simulink model "MMC_phase_hackathon_circuit1_HAAS_20260216"  (R2024b)
settings: Solver=FixedStepDiscrete  StartTime=t_init_sim  StopTime=sim_time  FixedStep=Ts  RelTol=1e-3
values from neighbouring files (symbols this model uses):
  a = 1    [param_phase_circuit1_20260216.m]
  C1low1_active = 1    [script_MMC_phase_circuit1_twist_20260216.m]
  C2low1_active = 1    [script_MMC_phase_circuit1_twist_20260216.m]
  C_M_extra = C_m-twist_high_side_C    [param_phase_circuit1_20260216.m]
  duty_cycle = 0.95    [script_MMC_phase_circuit1_twist_20260216.m]
  f0 = 50    [param_phase_circuit1_20260216.m]
  feeder_current_lower_rate_limit = -10    [script_MMC_phase_circuit1_twist_20260216.m]    (also in twist_parameters.m = -500)
  feeder_current_tab = [0.328 0.217 0.162 0.132 0.109 0.094 0.083 0.075 0.068 0.062 0.058 0.054 ... (42 elements, 14x3)]    [feeder_current.mat]
  feeder_current_upper_rate_limit = 0.386/(20e-3)    (= 19.3)    [twist_parameters.m]
  is6VExternallySupplied = true    [script_MMC_phase_circuit1_twist_20260216.m]
  isFeederJumperOpen = true    [script_MMC_phase_circuit1_twist_20260216.m]
  m = 1    [param_phase_circuit1_20260216.m]
  N = 5    [param_phase_circuit1_20260216.m]
  power_losses = false    [script_MMC_phase_circuit1_twist_20260216.m]
  source_V = 0    [script_MMC_phase_circuit1_twist_20260216.m]
  time_charge = 0.1    [script_MMC_phase_circuit1_twist_20260216.m]
  time_decharge = 0.6    [script_MMC_phase_circuit1_twist_20260216.m]
  Ts = 5e-7    (= 5e-07)    [script_MMC_phase_circuit1_twist_20260216.m]
  twist_data_acquisition_delay = 50e-9    (= 5e-08)    [script_MMC_phase_circuit1_twist_20260216.m]    (also in twist_parameters.m)
  twist_data_sampling_period = 1/twist_freq_data_sampling    (= 5e-05)    [script_MMC_phase_circuit1_twist_20260216.m]    (also in twist_parameters.m)
  twist_dead_time = 200e-9    (= 2e-07)    [twist_parameters.m]
  twist_freq_switching = 200e3    (= 200000)    [twist_parameters.m]
  twist_high_side_adc_R = 1/(1/2e6 + 1/2e6 + 1/(330e3+5.6e3))    (= 251272.836178)    [twist_parameters.m]
  twist_high_side_C = 33e-6*4 + 4.7e-6*12    (= 0.0001884)    [twist_parameters.m]
  twist_high_side_feeder_R = 47e3+4.7e3    (= 51700)    [twist_parameters.m]
  twist_high_side_rC = 0.1    [twist_parameters.m]
  twist_low_side_adc_R = 150e3+470    (= 150470)    [twist_parameters.m]
  twist_low_side_C_ceramic = 3*4.7e-6    (= 1.41e-05)    [twist_parameters.m]
  twist_low_side_C_electrolytic = 47e-6    (= 4.7e-05)    [twist_parameters.m]
  twist_low_side_L = 33e-6    (= 3.3e-05)    [twist_parameters.m]
  twist_low_side_rC = 700e-3    (= 0.7)    [twist_parameters.m]
  twist_low_side_rL = 20e-3    (= 0.02)    [twist_parameters.m]
  twist_R_VCC = (tau_VCC/twist_high_side_C  - twist_high_side_rC)/(1-(tau_VCC/twist_high_side_C - twist_high_side_rC)/R_parallel)    (= 1110.74997822)    [twist_parameters.m]
  VDC = 48    [param_phase_circuit1_20260216.m]
undefined symbols (not defined in the file or in its folder): feeder_current, gcbh, sps_rtmsupport, twist_low_side_lC
libraries: spsSeriesRLCBranchLib x130, spsTriangleGeneratorLib x60, spsMosfetLib x60, spsVoltageMeasurementLib x55, spsCurrentMeasurementLib x42, spsControlledCurrentSourceLib x30, spsDiodeLib x22, spsIdealSwitchLib x20, spsControlledVoltageSourceLib x2, spsGroundLib x1, spsMeanLib x1, spspowerguiLib x1
(part 1 of 18)
settings Model: Creator=ana  LastModifiedBy=ana

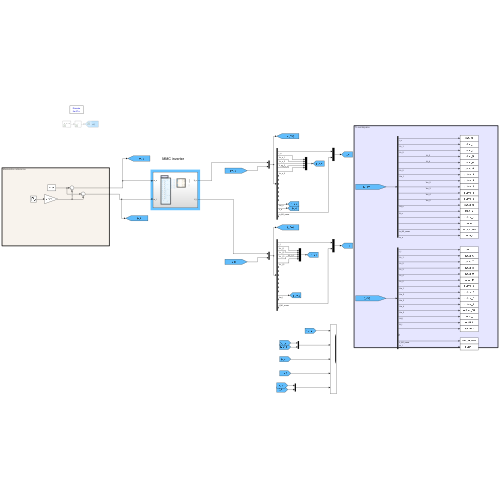
[thumbnail: Simulink's stored preview of the top-level diagram]
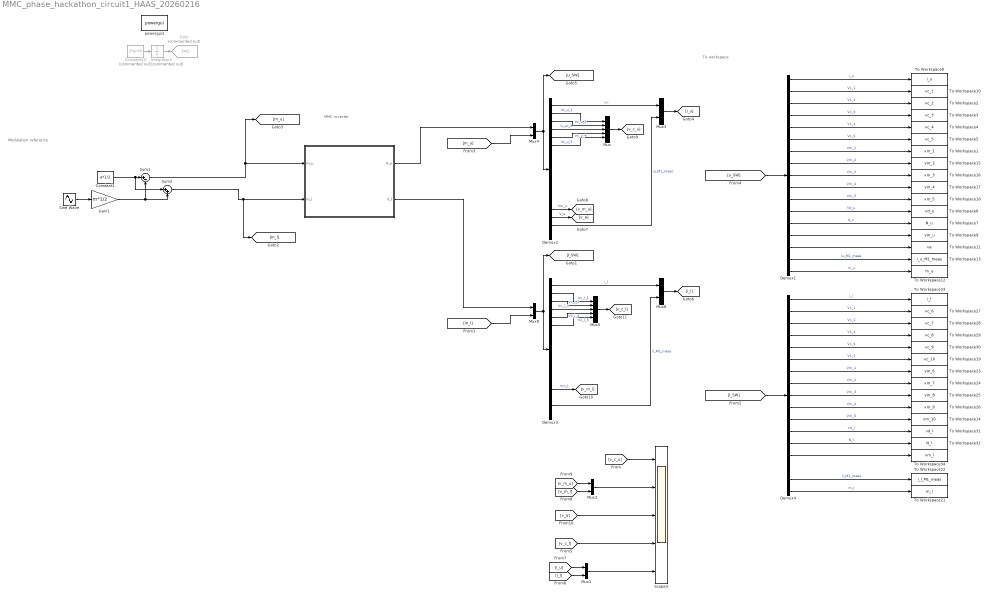
== system MMC_phase_hackathon_circuit1_HAAS_20260216 ==
  note: MMC inverter
  note: To workspace
  note: Modulation reference
  " " : Subsystem
  Constant1 : Constant  Value=a*1/2
  Constant12 : Constant  Commented=on  Value=2*pi*f0
  Demux{1..4} (4 alike) : Demux  Outputs=17
  Gain1 : Gain  Gain=m*1/2
  Goto : Goto  Commented=on  GotoTag=wt
  Integrator2 : Integrator  Commented=on
  Mux : Mux  Inputs=5
  Mux{1..4,8..9} (6 alike) : Mux  Inputs=2
  Mux5 : Mux  Inputs=5
  Scope3 : Scope  NumInputPorts=5
  Sine Wave : Sin  Frequency=2*pi*f0  SampleTime=Ts
  Sum1 : Sum  Inputs=|+-
  Sum2 : Sum  Inputs=|++
  To Workspace1 : ToWorkspace  VariableName=vm_1  SaveFormat=Structure With Time  SampleTime=-1
  To Workspace10 : ToWorkspace  VariableName=vc_1  SaveFormat=Structure With Time  SampleTime=-1
  To Workspace11 : ToWorkspace  VariableName=va  SaveFormat=Structure With Time  SampleTime=-1
  To Workspace12 : ToWorkspace  VariableName=m_u  SaveFormat=Structure With Time  SampleTime=-1
  To Workspace13 : ToWorkspace  VariableName=i_u_M1_meas  SaveFormat=Structure With Time  SampleTime=-1
  To Workspace14 : ToWorkspace  VariableName=vm_10  SaveFormat=Structure With Time  SampleTime=-1
  To Workspace15 : ToWorkspace  VariableName=vm_2  SaveFormat=Structure With Time  SampleTime=-1
  To Workspace16 : ToWorkspace  VariableName=vm_3  SaveFormat=Structure With Time  SampleTime=-1
  To Workspace17 : ToWorkspace  VariableName=vm_4  SaveFormat=Structure With Time  SampleTime=-1
  To Workspace18 : ToWorkspace  VariableName=vm_5  SaveFormat=Structure With Time  SampleTime=-1
  To Workspace19 : ToWorkspace  VariableName=vc_10  SaveFormat=Structure With Time  SampleTime=-1
  To Workspace2 : ToWorkspace  VariableName=vc_2  SaveFormat=Structure With Time  SampleTime=-1
  To Workspace21 : ToWorkspace  VariableName=m_l  SaveFormat=Structure With Time  SampleTime=-1
  To Workspace22 : ToWorkspace  VariableName=i_l_M1_meas  SaveFormat=Structure With Time  SampleTime=-1
  To Workspace23 : ToWorkspace  VariableName=vm_6  SaveFormat=Structure With Time  SampleTime=-1
  To Workspace24 : ToWorkspace  VariableName=vm_7  SaveFormat=Structure With Time  SampleTime=-1
  To Workspace25 : ToWorkspace  VariableName=vm_8  SaveFormat=Structure With Time  SampleTime=-1
  To Workspace26 : ToWorkspace  VariableName=vm_9  SaveFormat=Structure With Time  SampleTime=-1
  To Workspace27 : ToWorkspace  VariableName=vc_6  SaveFormat=Structure With Time  SampleTime=-1
  To Workspace28 : ToWorkspace  VariableName=vc_7  SaveFormat=Structure With Time  SampleTime=-1
  To Workspace29 : ToWorkspace  VariableName=vc_8  SaveFormat=Structure With Time  SampleTime=-1
  To Workspace3 : ToWorkspace  VariableName=vc_3  SaveFormat=Structure With Time  SampleTime=-1
  To Workspace30 : ToWorkspace  VariableName=vc_9  SaveFormat=Structure With Time  SampleTime=-1
  To Workspace31 : ToWorkspace  VariableName=vd_l  SaveFormat=Structure With Time  SampleTime=-1
  To Workspace32 : ToWorkspace  VariableName=N_l  SaveFormat=Structure With Time  SampleTime=-1
  To Workspace33 : ToWorkspace  VariableName=i_l  SaveFormat=Structure With Time  SampleTime=-1
  To Workspace34 : ToWorkspace  VariableName=vm_l  SaveFormat=Structure With Time  SampleTime=-1
  To Workspace4 : ToWorkspace  VariableName=vc_4  SaveFormat=Structure With Time  SampleTime=-1
  To Workspace5 : ToWorkspace  VariableName=vc_5  SaveFormat=Structure With Time  SampleTime=-1
  To Workspace6 : ToWorkspace  VariableName=vd_u  SaveFormat=Structure With Time  SampleTime=-1
  To Workspace7 : ToWorkspace  VariableName=N_u  SaveFormat=Structure With Time  SampleTime=-1
  To Workspace8 : ToWorkspace  VariableName=i_u  SaveFormat=Structure With Time  SampleTime=-1
  To Workspace9 : ToWorkspace  VariableName=vm_u  SaveFormat=Structure With Time  SampleTime=-1
  powergui1 : spspowerguiLib/powergui  Priority=1  SimulationMode=Discrete  SampleTime=Ts  frequency=60  Iterations=50  frequencyindice=0  Pbase=100e6  ErrMax=1e-4  UnitsV=V  UnitsW=W  buscounter=0  FunctionMessages=off  echomessages=off  EnableUseOfTLC=off  CurrentSourceSwitches=off  DisableSnubberDevices=off  DisableRonSwitches=off  DisableVfSwitches=off  DisplayEquations=off  AutomaticDiscreteSolvers=off  SolverType=Backward Euler  Interpol=off  ExternalGateDelay=off  methode=off  Ts=0  x0status=blocks  SPID=off  SwTol=0  HookPort=off  NonlinearTolerance=1e-4  nMaxIteration=100  ContinueOnMaxIteration=off  RestoreLinks=warning  ResistiveCurrentMeasurement=off  Frange=[0:2:500]  Ylog=off  Xlog=on  ShowGrid=off  save=off  variable=ZData  structure=0  ZoomFFT=off  StartTime=0.0  cycles=1  DisplayStyle=1  fundamental=60  FreqAxis=off  MaxFrequency=1000  frequencyindicesteady=1  RmsSteady=1  display=off
  wires:
  [u_SW] -> Demux1/1
  Demux1/8 -> To Workspace15/1  "Vm_2"
  Demux1/17 -> To Workspace12/1  "m_u"
  Demux1/10 -> To Workspace17/1  "Vm_4"
  Demux1/5 -> To Workspace4/1  "Vc_4"
  Demux1/12 -> To Workspace6/1  "Vd_u"
  " "/1(X_u) -> Mux4/1
  Demux2/1 -> Mux3/1  "i_u"
  Constant1/1 -> Sum2/1, Sum1/1
  Demux1/11 -> To Workspace18/1  "Vm_5"
  [m_u] -> Mux4/2
  Demux2/6 -> Mux/5  "Vc_u_5"
  Mux4/1 -> [u_SW], Demux2/1
  Constant12/1 -> Integrator2/1
  Integrator2/1 -> Goto/1
  Demux1/9 -> To Workspace16/1  "Vm_3"
  Demux1/7 -> To Workspace1/1  "Vm_1"
  Demux1/3 -> To Workspace2/1  "Vc_2"
  Demux1/4 -> To Workspace3/1  "Vc_3"
  Demux1/6 -> To Workspace5/1  "Vc_5"
  Gain1/1 -> Sum1/2, Sum2/2
  Demux1/2 -> To Workspace10/1  "Vc_1"
  Demux2/2 -> Mux/1  "Vc_u_1"
  Demux1/1 -> To Workspace8/1  "i_u"
  Demux2/5 -> Mux/4  "Vc_u_4"
  Demux2/3 -> Mux/2  "Vc_u_2"
  Demux2/4 -> Mux/3  "V_uc_3"
  Sum1/1 -> [m_u], " "/1(m_u)
  Demux2/14 -> [v_m_u]  "Vm_u"
  Sine Wave/1 -> Gain1/1
  Demux1/13 -> To Workspace7/1  "N_u"
  Demux1/14 -> To Workspace9/1
  Demux1/15 -> To Workspace11/1
  Demux2/16 -> Mux3/2  "iu_M1_meas"
  Demux1/16 -> To Workspace13/1  "iu_M1_meas"
  Sum2/1 -> [m_l], " "/2(m_l)
  Demux3/6 -> Mux5/5  "Vc_l_5"
  Mux8/1 -> [i_l]
  Mux9/1 -> [l_SW], Demux3/1
  Demux3/2 -> Mux5/1  "Vc_l_1"
  Demux3/3 -> Mux5/2  "Vc_l_2"
  Demux3/1 -> Mux8/1  "i_l"
  [m_l] -> Mux9/2
  " "/2(X_l) -> Mux9/1
  Demux3/14 -> [v_m_l]  "Vm_l"
  Demux3/16 -> Mux8/2  "il_M1_meas"
  Demux3/5 -> Mux5/4  "Vc_l_4"
  Demux3/4 -> Mux5/3  "Vc_l_3"
  Demux4/2 -> To Workspace27/1  "Vc_1"
  Demux4/12 -> To Workspace31/1  "Vd_l"
  Demux4/17 -> To Workspace21/1  "m_l"
  [l_SW] -> Demux4/1
  Demux4/1 -> To Workspace33/1  "i_l"
  Demux4/13 -> To Workspace32/1  "N_l"
  Demux4/14 -> To Workspace34/1
  Demux4/16 -> To Workspace22/1  "il_M1_meas"
  Demux4/3 -> To Workspace28/1  "Vc_2"
  Demux4/4 -> To Workspace29/1  "Vc_3"
  Demux4/5 -> To Workspace30/1  "Vc_4"
  Demux4/6 -> To Workspace19/1  "Vc_5"
  Demux4/7 -> To Workspace23/1  "Vm_1"
  Demux4/8 -> To Workspace24/1  "Vm_2"
  Demux4/9 -> To Workspace25/1  "Vm_3"
  Demux4/10 -> To Workspace26/1  "Vm_4"
  Demux4/11 -> To Workspace14/1  "Vm_5"
  Mux3/1 -> [i_u]
  Demux2/15 -> [v_a]  "V_a"
  Mux/1 -> [v_c_u]
  Mux5/1 -> [v_c_l]
  [v_c_u] -> Scope3/1
  [i_u] -> Mux1/1
  [i_l] -> Mux1/2
  [v_m_u] -> Mux2/1
  [v_m_l] -> Mux2/2
  [v_a] -> Scope3/3
  Mux2/1 -> Scope3/2
  Mux1/1 -> Scope3/5
  [v_c_l] -> Scope3/4

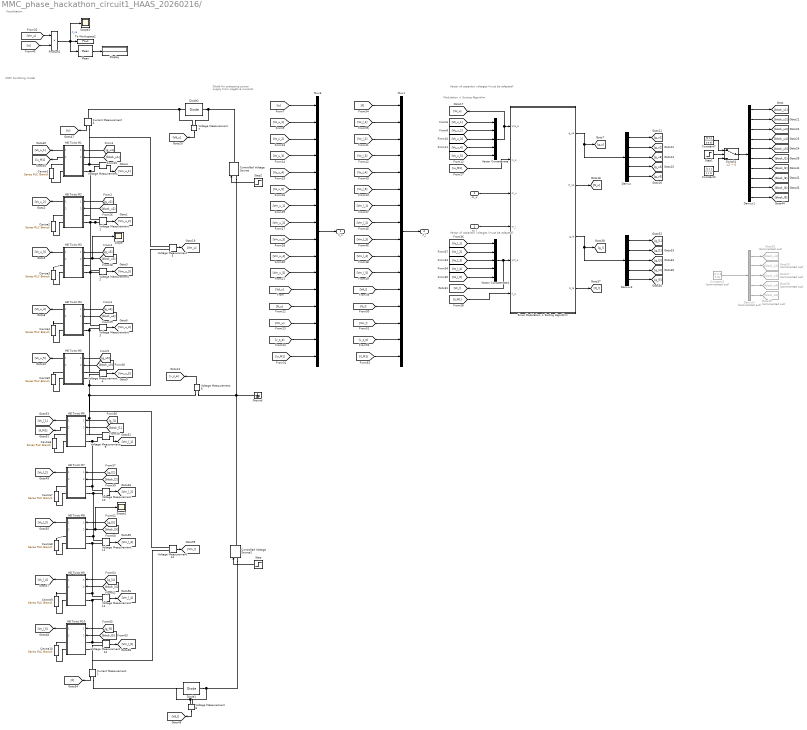
== system MMC_phase_hackathon_circuit1_HAAS_20260216/  ==
  note: Vector of capacitor voltages (must be adapted)
  note: Visualisation
  note: Modulation + Sorting Algorithm
  note: MMC Switching model
  note: Diode for protecting power supply from negative currents
  note: Vector of capacitor voltages (must be adapted)
  m_u : Inport
  m_l : Inport  Port=2
  Cextra{1..10} (10 alike) : spsSeriesRLCBranchLib/Series RLC Branch  LConnTagsString=__new0  RConnTagsString=__new0  BranchType=C  Resistance=twist_high_side_rC  Inductance=1e-3  SetiL0=off  InitialCurrent=0  Capacitance=C_M_extra  Setx0=on  InitialVoltage=source_V  Measurements=None
  Constant2 : Constant  Value=[1 1 1 1 1 1 1 1 1 1]
  Constant3 : Constant  Commented=on  Value=[0 0 0 0 0]
  Constant7 : Constant  Value=[0 0 0 0 0 0 0 0 0 0]
  Controlled Voltage Source : spsControlledVoltageSourceLib/Controlled Voltage Source  Initialize=on  Source_Type=DC  Amplitude=0  Phase=0  Frequency=0  Measurements=None
  Controlled Voltage Source1 : spsControlledVoltageSourceLib/Controlled Voltage Source  Initialize=on  Source_Type=DC  Amplitude=0  Phase=0  Frequency=0  Measurements=None
  Current Measurement1 : spsCurrentMeasurementLib/Current Measurement  PhasorSimulation=off  OutputType=Complex  PSBequivalent=0
  Current Measurement4 : spsCurrentMeasurementLib/Current Measurement  PhasorSimulation=off  OutputType=Complex  PSBequivalent=0
  Demux : Demux  Outputs=5
  Demux1 : Demux  Outputs=10
  Demux2 : Demux  Commented=on  Outputs=5
  Demux3 : Demux  Outputs=5
  Diode1 : spsDiodeLib/Diode  Ron=0.001  Lon=0  Vf=0.8  IC=0  UseSnubber=0  Rs=1e5  Cs=inf  Measurements=off
  Diode2 : spsDiodeLib/Diode  Ron=0.001  Lon=0  Vf=0.8  IC=0  UseSnubber=0  Rs=1e5  Cs=inf  Measurements=off
  Display : Display
  Goto25 : Goto  Commented=on  GotoTag=block_u1
  Goto26 : Goto  Commented=on  GotoTag=block_u2
  Goto27 : Goto  Commented=on  GotoTag=block_u3
  Goto28 : Goto  Commented=on  GotoTag=block_u4
  Goto29 : Goto  Commented=on  GotoTag=block_u5
  Ground : spsGroundLib/Ground  LConnTagsString=a
  HB Twist M1 : Subsystem
  HB Twist M10 : Subsystem
  HB Twist M2 : Subsystem
  HB Twist M3 : Subsystem
  HB Twist M4 : Subsystem
  HB Twist M5 : Subsystem
  HB Twist M6 : Subsystem
  HB Twist M7 : Subsystem
  HB Twist M8 : Subsystem
  HB Twist M9 : Subsystem
  Mean : spsMeanLib/Mean  Freq=f0  Vinit=0  Ts=Ts
  Mux1 : Mux  Inputs=16
  Mux6 : Mux  Inputs=16
  Product1 : Product
  Scope : Scope
  Scope1 : Scope
  Scope3 : Scope
  Sinus Modulation + Sorting Algorithm : Subsystem
  Step : Step  Time=time_decharge  Before=VDC/2  After=0  SampleTime=0
  Step1 : Step  Time=time_charge  SampleTime=Ts
  Step2 : Step  Time=time_decharge  Before=VDC/2  After=0  SampleTime=0
  Switch1 : Switch  Criteria=u2 > Threshold  SaturateOnIntegerOverflow=off  InputSameDT=off
  To Workspace2 : ToWorkspace  VariableName=Pout  SaveFormat=Structure With Time  SampleTime=-1
  Vector Concatenate : Concatenate  NumInputs=5
  Vector Concatenate1 : Concatenate  NumInputs=5
  Voltage Measurement{,1..14} (15 alike) : spsVoltageMeasurementLib/Voltage Measurement  PhasorSimulation=off  OutputType=Complex  PSBequivalent=0
  X_u : Outport
  X_l : Outport  Port=2
  wires:
  [Vc_u_1] -> Mux6/2
  Mux6/1 -> X_u/1
  Current Measurement4/1 -> [iu]
  Sinus Modulation + Sorting Algorithm/1(g_ua) -> Demux/1, [g_u]
  [iu_M1] -> Sinus Modulation + Sorting Algorithm/2(iu_a)
  Vector Concatenate/1 -> [Vc_u], Sinus Modulation + Sorting Algorithm/1(Vcu_a)
  m_u/1 -> Sinus Modulation + Sorting Algorithm/3(m_u)
  Product1/1 -> Mean/1, Scope3/1, To Workspace2/1  "P_sa"
  Voltage Measurement6/1 -> [v_s_a]
  [iu] -> Product1/2
  HB Twist M1/1(v_High) -> [Vc_u_1]
  Voltage Measurement/1 -> [Vm_u_1]
  [g_u1] -> HB Twist M1/1(duty_cycle1)
  Voltage Measurement1/1 -> [Vm_u_2]
  HB Twist M2/1(v_High) -> [Vc_u_2]
  [g_u2] -> HB Twist M2/1(duty_cycle1)
  [g_u3] -> HB Twist M3/1(duty_cycle1)
  HB Twist M3/1(v_High) -> [Vc_u_3]
  Voltage Measurement2/1 -> [Vm_u_3]
  [g_u4] -> HB Twist M4/1(duty_cycle1)
  HB Twist M4/1(v_High) -> [Vc_u_4]
  Voltage Measurement3/1 -> [Vm_u_4]
  [g_u5] -> HB Twist M5/1(duty_cycle1)
  HB Twist M5/1(v_High) -> [Vc_u_5]
  Voltage Measurement4/1 -> [Vm_u_5]
  [Vc_u_1] -> Vector Concatenate/1
  [Vc_u_2] -> Vector Concatenate/2
  [Vc_u_3] -> Vector Concatenate/3
  [Vc_u_4] -> Vector Concatenate/4
  [Vc_u_5] -> Vector Concatenate/5
  Demux/1 -> [g_u1]
  Demux/2 -> [g_u2]
  Demux/3 -> [g_u3]
  Demux/4 -> [g_u4]
  Demux/5 -> [g_u5]
  [iu] -> Mux6/1
  [Vc_u_2] -> Mux6/3
  [Vc_u_3] -> Mux6/4
  [Vc_u_4] -> Mux6/5
  [Vc_u_5] -> Mux6/6
  [Vm_u_1] -> Mux6/7
  [Vm_u_2] -> Mux6/8
  [Vm_u_3] -> Mux6/9
  [Vm_u_4] -> Mux6/10
  [Vm_u_5] -> Mux6/11
  [Vd_u] -> Mux6/12
  Sinus Modulation + Sorting Algorithm/2(N_ua) -> [N_u]
  [N_u] -> Mux6/13
  Voltage Measurement5/1 -> [Vm_u]
  [Vm_u] -> Mux6/14
  [v_s_a] -> Mux6/15
  Voltage Measurement7/1 -> [Vd_u]
  Mean/1 -> Display/1
  [block_u1] -> HB Twist M1/2(block_leg1)
  [block_u2] -> HB Twist M2/2(block_leg1)
  [block_u3] -> HB Twist M3/2(block_leg1), Scope/1
  [block_u4] -> HB Twist M4/2(block_leg1)
  [block_u5] -> HB Twist M5/2(block_leg1)
  Step1/1 -> Switch1/2
  Switch1/1 -> Demux1/1
  Demux1/1 -> [block_u1]
  Demux1/2 -> [block_u2]
  Demux1/3 -> [block_u3]
  Demux1/4 -> [block_u4]
  Demux1/5 -> [block_u5]
  Constant7/1 -> Switch1/1
  Constant2/1 -> Switch1/3
  Demux2/3 -> Goto27/1
  Demux2/4 -> Goto28/1
  Constant3/1 -> Demux2/1
  Demux2/5 -> Goto29/1
  Demux2/2 -> Goto26/1
  Demux2/1 -> Goto25/1
  HB Twist M1/2(i_1Low) -> [iu_M1]
  [iu_M1] -> Mux6/16
  [Vm_u] -> Product1/1
  m_l/1 -> Sinus Modulation + Sorting Algorithm/4(m_l)
  Vector Concatenate1/1 -> Sinus Modulation + Sorting Algorithm/5(Vcl_a), [Vc_l]
  [Vc_l_1] -> Vector Concatenate1/1
  [Vc_l_2] -> Vector Concatenate1/2
  [Vc_l_3] -> Vector Concatenate1/3
  [Vc_l_4] -> Vector Concatenate1/4
  [Vc_l_5] -> Vector Concatenate1/5
  [il_M1] -> Sinus Modulation + Sorting Algorithm/6(il_a)
  Sinus Modulation + Sorting Algorithm/3(g_la) -> Demux3/1, [g_l]
  Demux3/4 -> [g_l4]
  Demux3/3 -> [g_l3]
  Demux3/5 -> [g_l5]
  Demux3/2 -> [g_l2]
  Sinus Modulation + Sorting Algorithm/4(N_la) -> [N_l]
  Demux3/1 -> [g_l1]
  Demux1/6 -> [block_l1]
  Demux1/7 -> [block_l2]
  Demux1/8 -> [block_l3]
  Demux1/9 -> [block_l4]
  Demux1/10 -> [block_l5]
  [il] -> Mux1/1
  [Vc_l_5] -> Mux1/6
  [Vc_l_1] -> Mux1/2
  Mux1/1 -> X_l/1
  [Vm_l_4] -> Mux1/10
  [Vc_l_4] -> Mux1/5
  [Vm_l_2] -> Mux1/8
  [Vm_l_5] -> Mux1/11
  [il_M1] -> Mux1/16
  [Vc_l_2] -> Mux1/3
  [Vd_l] -> Mux1/12
  [Vm_l_1] -> Mux1/7
  [Vm_l_3] -> Mux1/9
  [Vm_l] -> Mux1/14
  [Vc_l_3] -> Mux1/4
  [N_l] -> Mux1/13
  [v_s_a] -> Mux1/15
  Voltage Measurement8/1 -> [Vd_l]
  Step/1 -> Controlled Voltage Source1/1
  Voltage Measurement12/1 -> [Vm_l_4]
  HB Twist M8/1(v_High) -> [Vc_l_3]
  HB Twist M7/1(v_High) -> [Vc_l_2]
  [block_l2] -> HB Twist M7/2(block_leg1)
  [g_l1] -> HB Twist M6/1(duty_cycle1)
  Voltage Measurement11/1 -> [Vm_l_3]
  Current Measurement1/1 -> [il]
  [g_l3] -> HB Twist M8/1(duty_cycle1)
  HB Twist M10/1(v_High) -> [Vc_l_5]
  [g_l2] -> HB Twist M7/1(duty_cycle1)
  HB Twist M9/1(v_High) -> [Vc_l_4]
  [block_l5] -> HB Twist M10/2(block_leg1)
  [block_l3] -> HB Twist M8/2(block_leg1), Scope1/1
  Voltage Measurement9/1 -> [Vm_l_1]
  Voltage Measurement10/1 -> [Vm_l_2]
  HB Twist M6/1(v_High) -> [Vc_l_1]
  [g_l5] -> HB Twist M10/1(duty_cycle1)
  HB Twist M6/2(i_1Low) -> [il_M1]
  [block_l1] -> HB Twist M6/2(block_leg1)
  [g_l4] -> HB Twist M9/1(duty_cycle1)
  [block_l4] -> HB Twist M9/2(block_leg1)
  Voltage Measurement13/1 -> [Vm_l_5]
  Voltage Measurement14/1 -> [Vm_l]
  Step2/1 -> Controlled Voltage Source/1
  connections:
  Voltage Measurement/LConn1 -- Current Measurement4/RConn1 -- Voltage Measurement5/LConn1 -- HB Twist M1/LConn1
  Voltage Measurement7/LConn2 -- Diode2/RConn1 -- Current Measurement4/LConn1
  Voltage Measurement3/LConn2 -- HB Twist M4/LConn2 -- HB Twist M5/LConn1 -- Voltage Measurement4/LConn1
  HB Twist M1/LConn2 -- Voltage Measurement/LConn2 -- HB Twist M2/LConn1 -- Voltage Measurement1/LConn1
  Voltage Measurement2/LConn2 -- HB Twist M3/LConn2 -- HB Twist M4/LConn1 -- Voltage Measurement3/LConn1
  Voltage Measurement1/LConn2 -- HB Twist M2/LConn2 -- HB Twist M3/LConn1 -- Voltage Measurement2/LConn1
  Voltage Measurement8/LConn1 -- Diode1/LConn1 -- Current Measurement1/RConn1
  Voltage Measurement7/LConn1 -- Diode2/LConn1 -- Controlled Voltage Source/RConn1
  Cextra1/LConn1 -- HB Twist M1/RConn1
  HB Twist M1/RConn2 -- Cextra1/RConn1
  Cextra2/LConn1 -- HB Twist M2/RConn1
  HB Twist M2/RConn2 -- Cextra2/RConn1
  HB Twist M3/RConn1 -- Cextra3/LConn1
  HB Twist M3/RConn2 -- Cextra3/RConn1
  Cextra4/LConn1 -- HB Twist M4/RConn1
  HB Twist M4/RConn2 -- Cextra4/RConn1
  HB Twist M5/RConn1 -- Cextra5/LConn1
  HB Twist M5/RConn2 -- Cextra5/RConn1
  Controlled Voltage Source/LConn1 -- Controlled Voltage Source1/RConn1 -- Voltage Measurement6/LConn2 -- Ground/LConn1
  Controlled Voltage Source1/LConn1 -- Diode1/RConn1 -- Voltage Measurement8/LConn2
  Voltage Measurement4/LConn2 -- Voltage Measurement9/LConn1 -- HB Twist M6/LConn1 -- Voltage Measurement14/LConn1 -- Voltage Measurement6/LConn1 -- Voltage Measurement5/LConn2 -- HB Twist M5/LConn2
  Voltage Measurement13/LConn1 -- HB Twist M10/LConn1 -- Voltage Measurement12/LConn2 -- HB Twist M9/LConn2
  Voltage Measurement11/LConn1 -- HB Twist M8/LConn1 -- Voltage Measurement10/LConn2 -- HB Twist M7/LConn2
  Voltage Measurement10/LConn1 -- HB Twist M6/LConn2 -- Voltage Measurement9/LConn2 -- HB Twist M7/LConn1
  Voltage Measurement13/LConn2 -- Voltage Measurement14/LConn2 -- Current Measurement1/LConn1 -- HB Twist M10/LConn2
  Voltage Measurement12/LConn1 -- HB Twist M9/LConn1 -- Voltage Measurement11/LConn2 -- HB Twist M8/LConn2
  Cextra9/LConn1 -- HB Twist M9/RConn1
  Cextra6/LConn1 -- HB Twist M6/RConn1
  Cextra7/LConn1 -- HB Twist M7/RConn1
  HB Twist M6/RConn2 -- Cextra6/RConn1
  HB Twist M8/RConn1 -- Cextra8/LConn1
  HB Twist M7/RConn2 -- Cextra7/RConn1
  HB Twist M10/RConn2 -- Cextra10/RConn1
  HB Twist M8/RConn2 -- Cextra8/RConn1
  HB Twist M10/RConn1 -- Cextra10/LConn1
  HB Twist M9/RConn2 -- Cextra9/RConn1

== system MMC_phase_hackathon_circuit1_HAAS_20260216/ /HB Twist M1 ==
  duty_cycle1 : Inport
  block_leg1 : Inport  Port=2
  Constant10 : Constant  Value=C2low1_active
  Constant11 : Constant  Value=isFeederJumperOpen
  Constant2 : Constant  Value=feeder_current_tab
  Constant3 : Constant  Value=-0.1
  Constant4 : Constant  Value=is6VExternallySupplied
  Constant5 : Constant  Value=power_losses
  Constant8 : Constant
  Constant9 : Constant  Value=C1low1_active
  Gain : Gain  Gain=-1
  Saturation : Saturate  UpperLimit=1  LowerLimit=0
  Twist Power Block : Subsystem
  Voltage Measurement8 : spsVoltageMeasurementLib/Voltage Measurement  PhasorSimulation=off  OutputType=Complex  PSBequivalent=0
  Load leg1 : PMIOPort  Side=Left
  Load GND : PMIOPort  Port=2  Side=Left
  Vhigh + : PMIOPort  Port=3  Side=Right
  Vhigh GND : PMIOPort  Port=4  Side=Right
  v_High : Outport
  i_1Low : Outport  Port=2
  wires:
  duty_cycle1/1 -> Saturation/1, Twist Power Block/1(duty_cycle1)
  Twist Power Block/2(v1Meas) -> [v1Meas_twist]
  block_leg1/1 -> Twist Power Block/8(block_leg1)
  Constant4/1 -> Twist Power Block/10(is6VExternallySupplied)
  Constant5/1 -> Twist Power Block/7(powerLosses)
  Twist Power Block/1(i1Meas) -> Gain/1
  Twist Power Block/5(v2Meas) -> [v2Meas_twist]
  Constant10/1 -> Twist Power Block/5(C2low_active)
  Constant3/1 -> Twist Power Block/3(duty_cycle2)
  Constant11/1 -> Twist Power Block/11(isFeederJumperOpen)
  Twist Power Block/4(i2Meas) -> [i2Meas_twist]
  Twist Power Block/3(vHMeas) -> [vHMeas_twist]
  Constant9/1 -> Twist Power Block/4(C1low_active)
  Twist Power Block/9(Q2) -> [Q2]
  Constant2/1 -> Twist Power Block/6(feeder_current_tab)
  Twist Power Block/6(iHMeas) -> [iHMeas_twist]
  Twist Power Block/7(feeder_current) -> [feeder_current_twist]
  Constant8/1 -> Twist Power Block/9(block_leg2)
  Twist Power Block/8(Q1) -> [Q1]
  Voltage Measurement8/1 -> v_High/1, [Vc_M1]
  Saturation/1 -> Twist Power Block/2(duty_cycle1_bis)
  Gain/1 -> i_1Low/1, [i1Meas_twist]
  connections:
  Voltage Measurement8/LConn2 -- Vhigh GND/RConn1 -- Twist Power Block/RConn2
  Voltage Measurement8/LConn1 -- Vhigh +/RConn1 -- Twist Power Block/RConn1
  Twist Power Block/LConn3 -- Load GND/RConn1
  Load leg1/RConn1 -- Twist Power Block/LConn1

== system MMC_phase_hackathon_circuit1_HAAS_20260216/ /HB Twist M10 ==
  duty_cycle1 : Inport
  block_leg1 : Inport  Port=2
  Constant10 : Constant  Value=C2low1_active
  Constant11 : Constant  Value=isFeederJumperOpen
  Constant2 : Constant  Value=feeder_current_tab
  Constant3 : Constant  Value=-0.1
  Constant4 : Constant  Value=is6VExternallySupplied
  Constant5 : Constant  Value=power_losses
  Constant8 : Constant
  Constant9 : Constant  Value=C1low1_active
  Gain : Gain  Gain=-1
  Saturation : Saturate  UpperLimit=1  LowerLimit=0
  Twist Power Block : Subsystem
  Voltage Measurement8 : spsVoltageMeasurementLib/Voltage Measurement  PhasorSimulation=off  OutputType=Complex  PSBequivalent=0
  Load leg1 : PMIOPort  Side=Left
  Load GND : PMIOPort  Port=2  Side=Left
  Vhigh + : PMIOPort  Port=3  Side=Right
  Vhigh GND : PMIOPort  Port=4  Side=Right
  v_High : Outport
  i_1Low : Outport  Port=2
  wires:
  duty_cycle1/1 -> Saturation/1, Twist Power Block/1(duty_cycle1)
  Twist Power Block/2(v1Meas) -> [v1Meas_twist]
  block_leg1/1 -> Twist Power Block/8(block_leg1)
  Constant4/1 -> Twist Power Block/10(is6VExternallySupplied)
  Constant5/1 -> Twist Power Block/7(powerLosses)
  Twist Power Block/1(i1Meas) -> Gain/1
  Twist Power Block/5(v2Meas) -> [v2Meas_twist]
  Constant10/1 -> Twist Power Block/5(C2low_active)
  Constant3/1 -> Twist Power Block/3(duty_cycle2)
  Constant11/1 -> Twist Power Block/11(isFeederJumperOpen)
  Twist Power Block/4(i2Meas) -> [i2Meas_twist]
  Twist Power Block/3(vHMeas) -> [vHMeas_twist]
  Constant9/1 -> Twist Power Block/4(C1low_active)
  Twist Power Block/9(Q2) -> [Q2]
  Constant2/1 -> Twist Power Block/6(feeder_current_tab)
  Twist Power Block/6(iHMeas) -> [iHMeas_twist]
  Twist Power Block/7(feeder_current) -> [feeder_current_twist]
  Constant8/1 -> Twist Power Block/9(block_leg2)
  Twist Power Block/8(Q1) -> [Q1]
  Voltage Measurement8/1 -> v_High/1, [Vc_M1]
  Saturation/1 -> Twist Power Block/2(duty_cycle1_bis)
  Gain/1 -> i_1Low/1, [i1Meas_twist]
  connections:
  Voltage Measurement8/LConn2 -- Vhigh GND/RConn1 -- Twist Power Block/RConn2
  Voltage Measurement8/LConn1 -- Vhigh +/RConn1 -- Twist Power Block/RConn1
  Twist Power Block/LConn3 -- Load GND/RConn1
  Load leg1/RConn1 -- Twist Power Block/LConn1

== system MMC_phase_hackathon_circuit1_HAAS_20260216/ /HB Twist M2 ==
  duty_cycle1 : Inport
  block_leg1 : Inport  Port=2
  Constant10 : Constant  Value=C2low1_active
  Constant11 : Constant  Value=isFeederJumperOpen
  Constant2 : Constant  Value=feeder_current_tab
  Constant3 : Constant  Value=-0.1
  Constant4 : Constant  Value=is6VExternallySupplied
  Constant5 : Constant  Value=power_losses
  Constant8 : Constant
  Constant9 : Constant  Value=C1low1_active
  Gain : Gain  Gain=-1
  Saturation : Saturate  UpperLimit=1  LowerLimit=0
  Twist Power Block : Subsystem
  Voltage Measurement8 : spsVoltageMeasurementLib/Voltage Measurement  PhasorSimulation=off  OutputType=Complex  PSBequivalent=0
  Load leg1 : PMIOPort  Side=Left
  Load GND : PMIOPort  Port=2  Side=Left
  Vhigh + : PMIOPort  Port=3  Side=Right
  Vhigh GND : PMIOPort  Port=4  Side=Right
  v_High : Outport
  i_1Low : Outport  Port=2
  wires:
  duty_cycle1/1 -> Saturation/1, Twist Power Block/1(duty_cycle1)
  Twist Power Block/2(v1Meas) -> [v1Meas_twist]
  block_leg1/1 -> Twist Power Block/8(block_leg1)
  Constant4/1 -> Twist Power Block/10(is6VExternallySupplied)
  Constant5/1 -> Twist Power Block/7(powerLosses)
  Twist Power Block/1(i1Meas) -> Gain/1
  Twist Power Block/5(v2Meas) -> [v2Meas_twist]
  Constant10/1 -> Twist Power Block/5(C2low_active)
  Constant3/1 -> Twist Power Block/3(duty_cycle2)
  Constant11/1 -> Twist Power Block/11(isFeederJumperOpen)
  Twist Power Block/4(i2Meas) -> [i2Meas_twist]
  Twist Power Block/3(vHMeas) -> [vHMeas_twist]
  Constant9/1 -> Twist Power Block/4(C1low_active)
  Twist Power Block/9(Q2) -> [Q2]
  Constant2/1 -> Twist Power Block/6(feeder_current_tab)
  Twist Power Block/6(iHMeas) -> [iHMeas_twist]
  Twist Power Block/7(feeder_current) -> [feeder_current_twist]
  Constant8/1 -> Twist Power Block/9(block_leg2)
  Twist Power Block/8(Q1) -> [Q1]
  Voltage Measurement8/1 -> v_High/1, [Vc_M1]
  Saturation/1 -> Twist Power Block/2(duty_cycle1_bis)
  Gain/1 -> i_1Low/1, [i1Meas_twist]
  connections:
  Voltage Measurement8/LConn2 -- Vhigh GND/RConn1 -- Twist Power Block/RConn2
  Voltage Measurement8/LConn1 -- Vhigh +/RConn1 -- Twist Power Block/RConn1
  Twist Power Block/LConn3 -- Load GND/RConn1
  Load leg1/RConn1 -- Twist Power Block/LConn1

== system MMC_phase_hackathon_circuit1_HAAS_20260216/ /HB Twist M3 ==
  duty_cycle1 : Inport
  block_leg1 : Inport  Port=2
  Constant10 : Constant  Value=C2low1_active
  Constant11 : Constant  Value=isFeederJumperOpen
  Constant2 : Constant  Value=feeder_current_tab
  Constant3 : Constant  Value=-0.1
  Constant4 : Constant  Value=is6VExternallySupplied
  Constant5 : Constant  Value=power_losses
  Constant8 : Constant
  Constant9 : Constant  Value=C1low1_active
  Gain : Gain  Gain=-1
  Saturation : Saturate  UpperLimit=1  LowerLimit=0
  Twist Power Block : Subsystem
  Voltage Measurement8 : spsVoltageMeasurementLib/Voltage Measurement  PhasorSimulation=off  OutputType=Complex  PSBequivalent=0
  Load leg1 : PMIOPort  Side=Left
  Load GND : PMIOPort  Port=2  Side=Left
  Vhigh + : PMIOPort  Port=3  Side=Right
  Vhigh GND : PMIOPort  Port=4  Side=Right
  v_High : Outport
  i_1Low : Outport  Port=2
  wires:
  duty_cycle1/1 -> Saturation/1, Twist Power Block/1(duty_cycle1)
  Twist Power Block/2(v1Meas) -> [v1Meas_twist]
  block_leg1/1 -> Twist Power Block/8(block_leg1)
  Constant4/1 -> Twist Power Block/10(is6VExternallySupplied)
  Constant5/1 -> Twist Power Block/7(powerLosses)
  Twist Power Block/1(i1Meas) -> Gain/1
  Twist Power Block/5(v2Meas) -> [v2Meas_twist]
  Constant10/1 -> Twist Power Block/5(C2low_active)
  Constant3/1 -> Twist Power Block/3(duty_cycle2)
  Constant11/1 -> Twist Power Block/11(isFeederJumperOpen)
  Twist Power Block/4(i2Meas) -> [i2Meas_twist]
  Twist Power Block/3(vHMeas) -> [vHMeas_twist]
  Constant9/1 -> Twist Power Block/4(C1low_active)
  Twist Power Block/9(Q2) -> [Q2]
  Constant2/1 -> Twist Power Block/6(feeder_current_tab)
  Twist Power Block/6(iHMeas) -> [iHMeas_twist]
  Twist Power Block/7(feeder_current) -> [feeder_current_twist]
  Constant8/1 -> Twist Power Block/9(block_leg2)
  Twist Power Block/8(Q1) -> [Q1]
  Voltage Measurement8/1 -> v_High/1, [Vc_M1]
  Saturation/1 -> Twist Power Block/2(duty_cycle1_bis)
  Gain/1 -> i_1Low/1, [i1Meas_twist]
  connections:
  Voltage Measurement8/LConn2 -- Vhigh GND/RConn1 -- Twist Power Block/RConn2
  Voltage Measurement8/LConn1 -- Vhigh +/RConn1 -- Twist Power Block/RConn1
  Twist Power Block/LConn3 -- Load GND/RConn1
  Load leg1/RConn1 -- Twist Power Block/LConn1

== system MMC_phase_hackathon_circuit1_HAAS_20260216/ /HB Twist M4 ==
  duty_cycle1 : Inport
  block_leg1 : Inport  Port=2
  Constant10 : Constant  Value=C2low1_active
  Constant11 : Constant  Value=isFeederJumperOpen
  Constant2 : Constant  Value=feeder_current_tab
  Constant3 : Constant  Value=-0.1
  Constant4 : Constant  Value=is6VExternallySupplied
  Constant5 : Constant  Value=power_losses
  Constant8 : Constant
  Constant9 : Constant  Value=C1low1_active
  Gain : Gain  Gain=-1
  Saturation : Saturate  UpperLimit=1  LowerLimit=0
  Twist Power Block : Subsystem
  Voltage Measurement8 : spsVoltageMeasurementLib/Voltage Measurement  PhasorSimulation=off  OutputType=Complex  PSBequivalent=0
  Load leg1 : PMIOPort  Side=Left
  Load GND : PMIOPort  Port=2  Side=Left
  Vhigh + : PMIOPort  Port=3  Side=Right
  Vhigh GND : PMIOPort  Port=4  Side=Right
  v_High : Outport
  i_1Low : Outport  Port=2
  wires:
  duty_cycle1/1 -> Saturation/1, Twist Power Block/1(duty_cycle1)
  Twist Power Block/2(v1Meas) -> [v1Meas_twist]
  block_leg1/1 -> Twist Power Block/8(block_leg1)
  Constant4/1 -> Twist Power Block/10(is6VExternallySupplied)
  Constant5/1 -> Twist Power Block/7(powerLosses)
  Twist Power Block/1(i1Meas) -> Gain/1
  Twist Power Block/5(v2Meas) -> [v2Meas_twist]
  Constant10/1 -> Twist Power Block/5(C2low_active)
  Constant3/1 -> Twist Power Block/3(duty_cycle2)
  Constant11/1 -> Twist Power Block/11(isFeederJumperOpen)
  Twist Power Block/4(i2Meas) -> [i2Meas_twist]
  Twist Power Block/3(vHMeas) -> [vHMeas_twist]
  Constant9/1 -> Twist Power Block/4(C1low_active)
  Twist Power Block/9(Q2) -> [Q2]
  Constant2/1 -> Twist Power Block/6(feeder_current_tab)
  Twist Power Block/6(iHMeas) -> [iHMeas_twist]
  Twist Power Block/7(feeder_current) -> [feeder_current_twist]
  Constant8/1 -> Twist Power Block/9(block_leg2)
  Twist Power Block/8(Q1) -> [Q1]
  Voltage Measurement8/1 -> v_High/1, [Vc_M1]
  Saturation/1 -> Twist Power Block/2(duty_cycle1_bis)
  Gain/1 -> i_1Low/1, [i1Meas_twist]
  connections:
  Voltage Measurement8/LConn2 -- Vhigh GND/RConn1 -- Twist Power Block/RConn2
  Voltage Measurement8/LConn1 -- Vhigh +/RConn1 -- Twist Power Block/RConn1
  Twist Power Block/LConn3 -- Load GND/RConn1
  Load leg1/RConn1 -- Twist Power Block/LConn1

== system MMC_phase_hackathon_circuit1_HAAS_20260216/ /HB Twist M5 ==
  duty_cycle1 : Inport
  block_leg1 : Inport  Port=2
  Constant10 : Constant  Value=C2low1_active
  Constant11 : Constant  Value=isFeederJumperOpen
  Constant2 : Constant  Value=feeder_current_tab
  Constant3 : Constant  Value=-0.1
  Constant4 : Constant  Value=is6VExternallySupplied
  Constant5 : Constant  Value=power_losses
  Constant8 : Constant
  Constant9 : Constant  Value=C1low1_active
  Gain : Gain  Gain=-1
  Saturation : Saturate  UpperLimit=1  LowerLimit=0
  Twist Power Block : Subsystem
  Voltage Measurement8 : spsVoltageMeasurementLib/Voltage Measurement  PhasorSimulation=off  OutputType=Complex  PSBequivalent=0
  Load leg1 : PMIOPort  Side=Left
  Load GND : PMIOPort  Port=2  Side=Left
  Vhigh + : PMIOPort  Port=3  Side=Right
  Vhigh GND : PMIOPort  Port=4  Side=Right
  v_High : Outport
  i_1Low : Outport  Port=2
  wires:
  duty_cycle1/1 -> Saturation/1, Twist Power Block/1(duty_cycle1)
  Twist Power Block/2(v1Meas) -> [v1Meas_twist]
  block_leg1/1 -> Twist Power Block/8(block_leg1)
  Constant4/1 -> Twist Power Block/10(is6VExternallySupplied)
  Constant5/1 -> Twist Power Block/7(powerLosses)
  Twist Power Block/1(i1Meas) -> Gain/1
  Twist Power Block/5(v2Meas) -> [v2Meas_twist]
  Constant10/1 -> Twist Power Block/5(C2low_active)
  Constant3/1 -> Twist Power Block/3(duty_cycle2)
  Constant11/1 -> Twist Power Block/11(isFeederJumperOpen)
  Twist Power Block/4(i2Meas) -> [i2Meas_twist]
  Twist Power Block/3(vHMeas) -> [vHMeas_twist]
  Constant9/1 -> Twist Power Block/4(C1low_active)
  Twist Power Block/9(Q2) -> [Q2]
  Constant2/1 -> Twist Power Block/6(feeder_current_tab)
  Twist Power Block/6(iHMeas) -> [iHMeas_twist]
  Twist Power Block/7(feeder_current) -> [feeder_current_twist]
  Constant8/1 -> Twist Power Block/9(block_leg2)
  Twist Power Block/8(Q1) -> [Q1]
  Voltage Measurement8/1 -> v_High/1, [Vc_M1]
  Saturation/1 -> Twist Power Block/2(duty_cycle1_bis)
  Gain/1 -> i_1Low/1, [i1Meas_twist]
  connections:
  Voltage Measurement8/LConn2 -- Vhigh GND/RConn1 -- Twist Power Block/RConn2
  Voltage Measurement8/LConn1 -- Vhigh +/RConn1 -- Twist Power Block/RConn1
  Twist Power Block/LConn3 -- Load GND/RConn1
  Load leg1/RConn1 -- Twist Power Block/LConn1

== system MMC_phase_hackathon_circuit1_HAAS_20260216/ /HB Twist M6 ==
  duty_cycle1 : Inport
  block_leg1 : Inport  Port=2
  Constant10 : Constant  Value=C2low1_active
  Constant11 : Constant  Value=isFeederJumperOpen
  Constant2 : Constant  Value=feeder_current_tab
  Constant3 : Constant  Value=-0.1
  Constant4 : Constant  Value=is6VExternallySupplied
  Constant5 : Constant  Value=power_losses
  Constant8 : Constant
  Constant9 : Constant  Value=C1low1_active
  Gain : Gain  Gain=-1
  Saturation : Saturate  UpperLimit=1  LowerLimit=0
  Twist Power Block : Subsystem
  Voltage Measurement8 : spsVoltageMeasurementLib/Voltage Measurement  PhasorSimulation=off  OutputType=Complex  PSBequivalent=0
  Load leg1 : PMIOPort  Side=Left
  Load GND : PMIOPort  Port=2  Side=Left
  Vhigh + : PMIOPort  Port=3  Side=Right
  Vhigh GND : PMIOPort  Port=4  Side=Right
  v_High : Outport
  i_1Low : Outport  Port=2
  wires:
  duty_cycle1/1 -> Saturation/1, Twist Power Block/1(duty_cycle1)
  Twist Power Block/2(v1Meas) -> [v1Meas_twist]
  block_leg1/1 -> Twist Power Block/8(block_leg1)
  Constant4/1 -> Twist Power Block/10(is6VExternallySupplied)
  Constant5/1 -> Twist Power Block/7(powerLosses)
  Twist Power Block/1(i1Meas) -> Gain/1
  Twist Power Block/5(v2Meas) -> [v2Meas_twist]
  Constant10/1 -> Twist Power Block/5(C2low_active)
  Constant3/1 -> Twist Power Block/3(duty_cycle2)
  Constant11/1 -> Twist Power Block/11(isFeederJumperOpen)
  Twist Power Block/4(i2Meas) -> [i2Meas_twist]
  Twist Power Block/3(vHMeas) -> [vHMeas_twist]
  Constant9/1 -> Twist Power Block/4(C1low_active)
  Twist Power Block/9(Q2) -> [Q2]
  Constant2/1 -> Twist Power Block/6(feeder_current_tab)
  Twist Power Block/6(iHMeas) -> [iHMeas_twist]
  Twist Power Block/7(feeder_current) -> [feeder_current_twist]
  Constant8/1 -> Twist Power Block/9(block_leg2)
  Twist Power Block/8(Q1) -> [Q1]
  Voltage Measurement8/1 -> v_High/1, [Vc_M1]
  Saturation/1 -> Twist Power Block/2(duty_cycle1_bis)
  Gain/1 -> i_1Low/1, [i1Meas_twist]
  connections:
  Voltage Measurement8/LConn2 -- Vhigh GND/RConn1 -- Twist Power Block/RConn2
  Voltage Measurement8/LConn1 -- Vhigh +/RConn1 -- Twist Power Block/RConn1
  Twist Power Block/LConn3 -- Load GND/RConn1
  Load leg1/RConn1 -- Twist Power Block/LConn1

== system MMC_phase_hackathon_circuit1_HAAS_20260216/ /HB Twist M7 ==
  duty_cycle1 : Inport
  block_leg1 : Inport  Port=2
  Constant10 : Constant  Value=C2low1_active
  Constant11 : Constant  Value=isFeederJumperOpen
  Constant2 : Constant  Value=feeder_current_tab
  Constant3 : Constant  Value=-0.1
  Constant4 : Constant  Value=is6VExternallySupplied
  Constant5 : Constant  Value=power_losses
  Constant8 : Constant
  Constant9 : Constant  Value=C1low1_active
  Gain : Gain  Gain=-1
  Saturation : Saturate  UpperLimit=1  LowerLimit=0
  Twist Power Block : Subsystem
  Voltage Measurement8 : spsVoltageMeasurementLib/Voltage Measurement  PhasorSimulation=off  OutputType=Complex  PSBequivalent=0
  Load leg1 : PMIOPort  Side=Left
  Load GND : PMIOPort  Port=2  Side=Left
  Vhigh + : PMIOPort  Port=3  Side=Right
  Vhigh GND : PMIOPort  Port=4  Side=Right
  v_High : Outport
  i_1Low : Outport  Port=2
  wires:
  duty_cycle1/1 -> Saturation/1, Twist Power Block/1(duty_cycle1)
  Twist Power Block/2(v1Meas) -> [v1Meas_twist]
  block_leg1/1 -> Twist Power Block/8(block_leg1)
  Constant4/1 -> Twist Power Block/10(is6VExternallySupplied)
  Constant5/1 -> Twist Power Block/7(powerLosses)
  Twist Power Block/1(i1Meas) -> Gain/1
  Twist Power Block/5(v2Meas) -> [v2Meas_twist]
  Constant10/1 -> Twist Power Block/5(C2low_active)
  Constant3/1 -> Twist Power Block/3(duty_cycle2)
  Constant11/1 -> Twist Power Block/11(isFeederJumperOpen)
  Twist Power Block/4(i2Meas) -> [i2Meas_twist]
  Twist Power Block/3(vHMeas) -> [vHMeas_twist]
  Constant9/1 -> Twist Power Block/4(C1low_active)
  Twist Power Block/9(Q2) -> [Q2]
  Constant2/1 -> Twist Power Block/6(feeder_current_tab)
  Twist Power Block/6(iHMeas) -> [iHMeas_twist]
  Twist Power Block/7(feeder_current) -> [feeder_current_twist]
  Constant8/1 -> Twist Power Block/9(block_leg2)
  Twist Power Block/8(Q1) -> [Q1]
  Voltage Measurement8/1 -> v_High/1, [Vc_M1]
  Saturation/1 -> Twist Power Block/2(duty_cycle1_bis)
  Gain/1 -> i_1Low/1, [i1Meas_twist]
  connections:
  Voltage Measurement8/LConn2 -- Vhigh GND/RConn1 -- Twist Power Block/RConn2
  Voltage Measurement8/LConn1 -- Vhigh +/RConn1 -- Twist Power Block/RConn1
  Twist Power Block/LConn3 -- Load GND/RConn1
  Load leg1/RConn1 -- Twist Power Block/LConn1

== system MMC_phase_hackathon_circuit1_HAAS_20260216/ /HB Twist M8 ==
  duty_cycle1 : Inport
  block_leg1 : Inport  Port=2
  Constant10 : Constant  Value=C2low1_active
  Constant11 : Constant  Value=isFeederJumperOpen
  Constant2 : Constant  Value=feeder_current_tab
  Constant3 : Constant  Value=-0.1
  Constant4 : Constant  Value=is6VExternallySupplied
  Constant5 : Constant  Value=power_losses
  Constant8 : Constant
  Constant9 : Constant  Value=C1low1_active
  Gain : Gain  Gain=-1
  Saturation : Saturate  UpperLimit=1  LowerLimit=0
  Twist Power Block : Subsystem
  Voltage Measurement8 : spsVoltageMeasurementLib/Voltage Measurement  PhasorSimulation=off  OutputType=Complex  PSBequivalent=0
  Load leg1 : PMIOPort  Side=Left
  Load GND : PMIOPort  Port=2  Side=Left
  Vhigh + : PMIOPort  Port=3  Side=Right
  Vhigh GND : PMIOPort  Port=4  Side=Right
  v_High : Outport
  i_1Low : Outport  Port=2
  wires:
  duty_cycle1/1 -> Saturation/1, Twist Power Block/1(duty_cycle1)
  Twist Power Block/2(v1Meas) -> [v1Meas_twist]
  block_leg1/1 -> Twist Power Block/8(block_leg1)
  Constant4/1 -> Twist Power Block/10(is6VExternallySupplied)
  Constant5/1 -> Twist Power Block/7(powerLosses)
  Twist Power Block/1(i1Meas) -> Gain/1
  Twist Power Block/5(v2Meas) -> [v2Meas_twist]
  Constant10/1 -> Twist Power Block/5(C2low_active)
  Constant3/1 -> Twist Power Block/3(duty_cycle2)
  Constant11/1 -> Twist Power Block/11(isFeederJumperOpen)
  Twist Power Block/4(i2Meas) -> [i2Meas_twist]
  Twist Power Block/3(vHMeas) -> [vHMeas_twist]
  Constant9/1 -> Twist Power Block/4(C1low_active)
  Twist Power Block/9(Q2) -> [Q2]
  Constant2/1 -> Twist Power Block/6(feeder_current_tab)
  Twist Power Block/6(iHMeas) -> [iHMeas_twist]
  Twist Power Block/7(feeder_current) -> [feeder_current_twist]
  Constant8/1 -> Twist Power Block/9(block_leg2)
  Twist Power Block/8(Q1) -> [Q1]
  Voltage Measurement8/1 -> v_High/1, [Vc_M1]
  Saturation/1 -> Twist Power Block/2(duty_cycle1_bis)
  Gain/1 -> i_1Low/1, [i1Meas_twist]
  connections:
  Voltage Measurement8/LConn2 -- Vhigh GND/RConn1 -- Twist Power Block/RConn2
  Voltage Measurement8/LConn1 -- Vhigh +/RConn1 -- Twist Power Block/RConn1
  Twist Power Block/LConn3 -- Load GND/RConn1
  Load leg1/RConn1 -- Twist Power Block/LConn1

== system MMC_phase_hackathon_circuit1_HAAS_20260216/ /HB Twist M9 ==
  duty_cycle1 : Inport
  block_leg1 : Inport  Port=2
  Constant10 : Constant  Value=C2low1_active
  Constant11 : Constant  Value=isFeederJumperOpen
  Constant2 : Constant  Value=feeder_current_tab
  Constant3 : Constant  Value=-0.1
  Constant4 : Constant  Value=is6VExternallySupplied
  Constant5 : Constant  Value=power_losses
  Constant8 : Constant
  Constant9 : Constant  Value=C1low1_active
  Gain : Gain  Gain=-1
  Saturation : Saturate  UpperLimit=1  LowerLimit=0
  Twist Power Block : Subsystem
  Voltage Measurement8 : spsVoltageMeasurementLib/Voltage Measurement  PhasorSimulation=off  OutputType=Complex  PSBequivalent=0
  Load leg1 : PMIOPort  Side=Left
  Load GND : PMIOPort  Port=2  Side=Left
  Vhigh + : PMIOPort  Port=3  Side=Right
  Vhigh GND : PMIOPort  Port=4  Side=Right
  v_High : Outport
  i_1Low : Outport  Port=2
  wires:
  duty_cycle1/1 -> Saturation/1, Twist Power Block/1(duty_cycle1)
  Twist Power Block/2(v1Meas) -> [v1Meas_twist]
  block_leg1/1 -> Twist Power Block/8(block_leg1)
  Constant4/1 -> Twist Power Block/10(is6VExternallySupplied)
  Constant5/1 -> Twist Power Block/7(powerLosses)
  Twist Power Block/1(i1Meas) -> Gain/1
  Twist Power Block/5(v2Meas) -> [v2Meas_twist]
  Constant10/1 -> Twist Power Block/5(C2low_active)
  Constant3/1 -> Twist Power Block/3(duty_cycle2)
  Constant11/1 -> Twist Power Block/11(isFeederJumperOpen)
  Twist Power Block/4(i2Meas) -> [i2Meas_twist]
  Twist Power Block/3(vHMeas) -> [vHMeas_twist]
  Constant9/1 -> Twist Power Block/4(C1low_active)
  Twist Power Block/9(Q2) -> [Q2]
  Constant2/1 -> Twist Power Block/6(feeder_current_tab)
  Twist Power Block/6(iHMeas) -> [iHMeas_twist]
  Twist Power Block/7(feeder_current) -> [feeder_current_twist]
  Constant8/1 -> Twist Power Block/9(block_leg2)
  Twist Power Block/8(Q1) -> [Q1]
  Voltage Measurement8/1 -> v_High/1, [Vc_M1]
  Saturation/1 -> Twist Power Block/2(duty_cycle1_bis)
  Gain/1 -> i_1Low/1, [i1Meas_twist]
  connections:
  Voltage Measurement8/LConn2 -- Vhigh GND/RConn1 -- Twist Power Block/RConn2
  Voltage Measurement8/LConn1 -- Vhigh +/RConn1 -- Twist Power Block/RConn1
  Twist Power Block/LConn3 -- Load GND/RConn1
  Load leg1/RConn1 -- Twist Power Block/LConn1

== system MMC_phase_hackathon_circuit1_HAAS_20260216/ /Sinus Modulation + Sorting Algorithm ==
  note: Stack u
  note: Stack l
  Vcu_a : Inport
  iu_a : Inport  Port=2
  m_u : Inport  Port=3
  m_l : Inport  Port=4
  Vcl_a : Inport  Port=5
  il_a : Inport  Port=6
  Constant : Constant
  Constant1 : Constant  Value=0
  Constant2 : Constant
  Constant3 : Constant  Value=0
  GreaterThan : RelationalOperator  Operator=~=  OutDataTypeStr=boolean  RndMeth=Simplest  InputSameDT=off
  GreaterThan1 : RelationalOperator  Operator=~=  OutDataTypeStr=boolean  RndMeth=Simplest  InputSameDT=off
  Memory : Memory  InheritSampleTime=on  LinearizeMemory=on  LinearizeAsDelay=on
  Memory1 : Memory  InheritSampleTime=on  LinearizeMemory=on  LinearizeAsDelay=on
  Number_of_Module_to_SWITCH : Subsystem
  Subsystem1 : Subsystem
      settings: PortSchema="{\"entries\":[{\"content\":{\"sides\":[{\"content\":{\"connectorIds\":[\"In1\",\"In2\",\"In3\"]},\"type\":\"ConnectorPlacement.EquallySpacedRectSide\",\"uuid\":\"25566ff9-210a-4488-8b15-702d65e93a4b\"},{\"content\":{\"connectorIds\":[\"Out1\"],\"side\":\"RIGHT\"},\"type\":\"ConnectorPlacement.EquallySpacedRectSide\",\"uuid\":\"97373fc2-3782-4e65-8804-644d53fa5380\"},{\"content\":{\"connectorIds\":[\"In4\"],\"side\":\"TOP\"},\"type\":\"ConnectorPlacement.EquallySpacedRectSide\",\"uuid\":\"e65d2433-d029-4e4a-b081-22e9ded4f272\"}]},\"type\":\"ConnectorPlacement.EquallySpacedConnector\",\"uuid\":\"235c80e7-78ad-4e69-a231-ec76d675b4ae\"}],\"packageUris\":[\"http://schema.mathworks.com/mf0/Connector/R2020b\"],\"version\":\"1.0\"}"
  Subsystem2 : Subsystem
      settings: PortSchema="{\"entries\":[{\"content\":{\"sides\":[{\"content\":{\"connectorIds\":[\"In1\",\"In2\",\"In3\"]},\"type\":\"ConnectorPlacement.EquallySpacedRectSide\",\"uuid\":\"25566ff9-210a-4488-8b15-702d65e93a4b\"},{\"content\":{\"connectorIds\":[\"Out1\"],\"side\":\"RIGHT\"},\"type\":\"ConnectorPlacement.EquallySpacedRectSide\",\"uuid\":\"97373fc2-3782-4e65-8804-644d53fa5380\"},{\"content\":{\"connectorIds\":[\"In4\"],\"side\":\"TOP\"},\"type\":\"ConnectorPlacement.EquallySpacedRectSide\",\"uuid\":\"e65d2433-d029-4e4a-b081-22e9ded4f272\"}]},\"type\":\"ConnectorPlacement.EquallySpacedConnector\",\"uuid\":\"235c80e7-78ad-4e69-a231-ec76d675b4ae\"}],\"packageUris\":[\"http://schema.mathworks.com/mf0/Connector/R2020b\"],\"version\":\"1.0\"}"
  Switch : Switch  Criteria=u2 > Threshold  SaturateOnIntegerOverflow=off  InputSameDT=off
  Switch1 : Switch  Criteria=u2 > Threshold  SaturateOnIntegerOverflow=off  InputSameDT=off
  g_ua : Outport
  N_ua : Outport  Port=2
  g_la : Outport  Port=3
  N_la : Outport  Port=4
  wires:
  Vcu_a/1 -> Subsystem1/1(Vc_unitaire_stack)
  iu_a/1 -> Subsystem1/2(i_stack)
  Number_of_Module_to_SWITCH/1(Nu_a) -> Subsystem1/3(N_on_stack), GreaterThan/1, Memory/1, N_ua/1
  m_u/1 -> Number_of_Module_to_SWITCH/1(Modulante ua)
  Subsystem1/1(g_unitaire_stack) -> g_ua/1
  Switch/1 -> Subsystem1/4(Pulse)
  Memory/1 -> GreaterThan/2
  GreaterThan/1 -> Switch/2
  Constant/1 -> Switch/1
  Constant1/1 -> Switch/3
  m_l/1 -> Number_of_Module_to_SWITCH/2(Modulante la)
  GreaterThan1/1 -> Switch1/2
  Switch1/1 -> Subsystem2/4(Pulse)
  Memory1/1 -> GreaterThan1/2
  Constant2/1 -> Switch1/1
  Vcl_a/1 -> Subsystem2/1(Vc_unitaire_stack)
  Constant3/1 -> Switch1/3
  Number_of_Module_to_SWITCH/2(Nl_a) -> Subsystem2/3(N_on_stack), GreaterThan1/1, Memory1/1, N_la/1
  il_a/1 -> Subsystem2/2(i_stack)
  Subsystem2/1(g_unitaire_stack) -> g_la/1
